simulink model "MMC_stack_openloop_NLM_CVB_dutycycleramp_twist"  (R2024b)
settings: Solver=FixedStepDiscrete  StartTime=t_init_sim  StopTime=sim_time  FixedStep=Ts  RelTol=1e-3
values from neighbouring files (symbols this model uses):
  a = 1    [param_stacksim_20260219.m]
  C1low1_active = 1    [script_MMC_stack_dutycycleramp_twist_20260219.m]
  C2low1_active = 1    [script_MMC_stack_dutycycleramp_twist_20260219.m]
  C_M_extra = C_m-twist_high_side_C    [param_stacksim_20260219.m]
  duty_cycle_max = 0.95    [script_MMC_stack_dutycycleramp_twist_20260219.m]
  duty_cycle_min = 0    [script_MMC_stack_dutycycleramp_twist_20260219.m]
  f0 = 50    [param_stacksim_20260219.m]
  feeder_current_lower_rate_limit = -10    [script_MMC_stack_dutycycleramp_twist_20260219.m]    (also in twist_parameters.m = -500)
  feeder_current_tab = [0.328 0.217 0.162 0.132 0.109 0.094 0.083 0.075 0.068 0.062 0.058 0.054 ... (42 elements, 14x3)]    [feeder_current.mat]
  feeder_current_upper_rate_limit = 0.386/(20e-3)    (= 19.3)    [twist_parameters.m]
  is6VExternallySupplied = true    [script_MMC_stack_dutycycleramp_twist_20260219.m]
  isDutyCycleRamp = true    [script_MMC_stack_dutycycleramp_twist_20260219.m]
  isFeederJumperOpen = true    [script_MMC_stack_dutycycleramp_twist_20260219.m]
  L_arm = 30e-3    (= 0.03)    [param_stacksim_20260219.m]
  m = 1    [param_stacksim_20260219.m]
  N = 5    [param_stacksim_20260219.m]
  power_losses = false    [script_MMC_stack_dutycycleramp_twist_20260219.m]
  R = 30    [param_stacksim_20260219.m]
  ramp_step_time = 500    [script_MMC_stack_dutycycleramp_twist_20260219.m]
  ramp_ticks = 4    [script_MMC_stack_dutycycleramp_twist_20260219.m]
  source_V = 0    [script_MMC_stack_dutycycleramp_twist_20260219.m]
  time_charge = 0.2    [script_MMC_stack_dutycycleramp_twist_20260219.m]
  time_decharge = 0.8    [script_MMC_stack_dutycycleramp_twist_20260219.m]
  Ts = 5e-7    (= 5e-07)    [script_MMC_stack_dutycycleramp_twist_20260219.m]
  twist_dead_time = 200e-9    (= 2e-07)    [twist_parameters.m]
  twist_freq_switching = 200e3    (= 200000)    [twist_parameters.m]
  twist_high_side_adc_R = 1/(1/2e6 + 1/2e6 + 1/(330e3+5.6e3))    (= 251272.836178)    [twist_parameters.m]
  twist_high_side_C = 33e-6*4 + 4.7e-6*12    (= 0.0001884)    [twist_parameters.m]
  twist_high_side_feeder_R = 47e3+4.7e3    (= 51700)    [twist_parameters.m]
  twist_high_side_rC = 0.1    [twist_parameters.m]
  twist_low_side_adc_R = 150e3+470    (= 150470)    [twist_parameters.m]
  twist_low_side_C_ceramic = 3*4.7e-6    (= 1.41e-05)    [twist_parameters.m]
  twist_low_side_C_electrolytic = 47e-6    (= 4.7e-05)    [twist_parameters.m]
  twist_low_side_L = 33e-6    (= 3.3e-05)    [twist_parameters.m]
  twist_low_side_rC = 700e-3    (= 0.7)    [twist_parameters.m]
  twist_low_side_rL = 20e-3    (= 0.02)    [twist_parameters.m]
  twist_R_VCC = (tau_VCC/twist_high_side_C  - twist_high_side_rC)/(1-(tau_VCC/twist_high_side_C - twist_high_side_rC)/R_parallel)    (= 1110.74997822)    [twist_parameters.m]
  VDC = 48    [param_stacksim_20260219.m]
undefined symbols (not defined in the file or in its folder): C_SM, feeder_current, gcbh, sps_rtmsupport, twist_data_acquisition_delay, twist_data_sampling_period, twist_low_side_lC
libraries: spsSeriesRLCBranchLib x66, spsTriangleGeneratorLib x30, spsMosfetLib x30, spsVoltageMeasurementLib x30, spsCurrentMeasurementLib x21, spsControlledCurrentSourceLib x15, spsDiodeLib x11, spsIdealSwitchLib x10, spsControlledVoltageSourceLib x1, spsGroundLib x1, spsMeanLib x1, spspowerguiLib x1
(part 1 of 9)
settings Model: Creator=ana  LastModifiedBy=ana

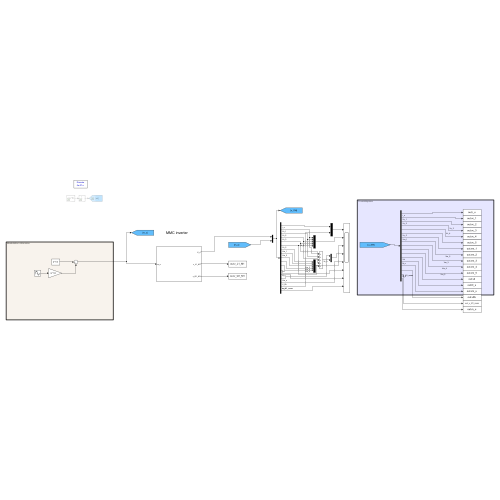
[thumbnail: Simulink's stored preview of the top-level diagram]
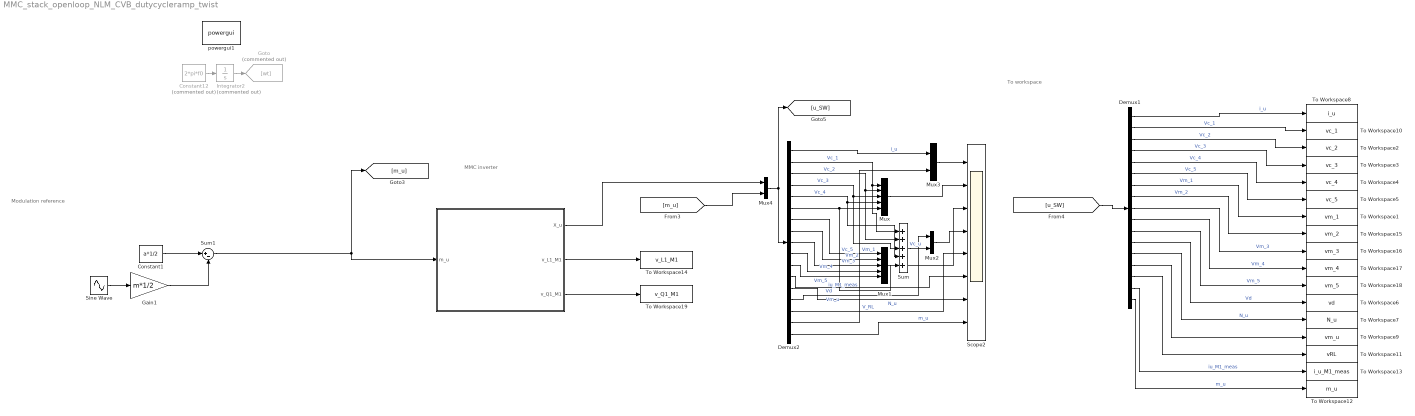
== system MMC_stack_openloop_NLM_CVB_dutycycleramp_twist ==
  note: MMC inverter
  note: To workspace
  note: Modulation reference
  " " : Subsystem
  Constant1 : Constant  Value=a*1/2
  Constant12 : Constant  Commented=on  Value=2*pi*f0
  Demux1 : Demux  Outputs=17
  Demux2 : Demux  Outputs=17
  Gain1 : Gain  Gain=m*1/2
  Goto : Goto  Commented=on  GotoTag=wt
  Integrator2 : Integrator  Commented=on
  Mux : Mux  Inputs=5
  Mux1 : Mux  Inputs=5
  Mux2 : Mux  Inputs=2
  Mux3 : Mux  Inputs=2
  Mux4 : Mux  Inputs=2
  Scope2 : Scope  NumInputPorts=8
  Sine Wave : Sin  Frequency=2*pi*f0  SampleTime=Ts
  Sum : Sum  Inputs=+++++
  Sum1 : Sum  Inputs=|+-
  To Workspace1 : ToWorkspace  VariableName=vm_1  SaveFormat=Structure With Time  SampleTime=-1
  To Workspace10 : ToWorkspace  VariableName=vc_1  SaveFormat=Structure With Time  SampleTime=-1
  To Workspace11 : ToWorkspace  VariableName=vRL  SaveFormat=Structure With Time  SampleTime=-1
  To Workspace12 : ToWorkspace  VariableName=m_u  SaveFormat=Structure With Time  SampleTime=-1
  To Workspace13 : ToWorkspace  VariableName=i_u_M1_meas  SaveFormat=Structure With Time  SampleTime=-1
  To Workspace14 : ToWorkspace  VariableName=v_L1_M1  SaveFormat=Structure With Time  SampleTime=-1
  To Workspace15 : ToWorkspace  VariableName=vm_2  SaveFormat=Structure With Time  SampleTime=-1
  To Workspace16 : ToWorkspace  VariableName=vm_3  SaveFormat=Structure With Time  SampleTime=-1
  To Workspace17 : ToWorkspace  VariableName=vm_4  SaveFormat=Structure With Time  SampleTime=-1
  To Workspace18 : ToWorkspace  VariableName=vm_5  SaveFormat=Structure With Time  SampleTime=-1
  To Workspace19 : ToWorkspace  VariableName=v_Q1_M1  SaveFormat=Structure With Time  SampleTime=-1
  To Workspace2 : ToWorkspace  VariableName=vc_2  SaveFormat=Structure With Time  SampleTime=-1
  To Workspace3 : ToWorkspace  VariableName=vc_3  SaveFormat=Structure With Time  SampleTime=-1
  To Workspace4 : ToWorkspace  VariableName=vc_4  SaveFormat=Structure With Time  SampleTime=-1
  To Workspace5 : ToWorkspace  VariableName=vc_5  SaveFormat=Structure With Time  SampleTime=-1
  To Workspace6 : ToWorkspace  VariableName=vd  SaveFormat=Structure With Time  SampleTime=-1
  To Workspace7 : ToWorkspace  VariableName=N_u  SaveFormat=Structure With Time  SampleTime=-1
  To Workspace8 : ToWorkspace  VariableName=i_u  SaveFormat=Structure With Time  SampleTime=-1
  To Workspace9 : ToWorkspace  VariableName=vm_u  SaveFormat=Structure With Time  SampleTime=-1
  powergui1 : spspowerguiLib/powergui  Priority=1  SimulationMode=Discrete  SampleTime=Ts  frequency=60  Iterations=50  frequencyindice=0  Pbase=100e6  ErrMax=1e-4  UnitsV=V  UnitsW=W  buscounter=0  FunctionMessages=off  echomessages=off  EnableUseOfTLC=off  CurrentSourceSwitches=off  DisableSnubberDevices=off  DisableRonSwitches=off  DisableVfSwitches=off  DisplayEquations=off  AutomaticDiscreteSolvers=off  SolverType=Backward Euler  Interpol=off  ExternalGateDelay=off  methode=off  Ts=0  x0status=blocks  SPID=off  SwTol=0  HookPort=off  NonlinearTolerance=1e-4  nMaxIteration=100  ContinueOnMaxIteration=off  RestoreLinks=warning  ResistiveCurrentMeasurement=off  Frange=[0:2:500]  Ylog=off  Xlog=on  ShowGrid=off  save=off  variable=ZData  structure=0  ZoomFFT=off  StartTime=0.0  cycles=1  DisplayStyle=1  fundamental=60  FreqAxis=off  MaxFrequency=1000  frequencyindicesteady=1  RmsSteady=1  display=off
  wires:
  Demux2/7 -> Mux1/1  "Vm_1"
  Demux2/11 -> Mux1/5  "Vm_5"
  Demux2/9 -> Mux1/3  "Vm_3"
  [u_SW] -> Demux1/1
  Demux1/8 -> To Workspace15/1  "Vm_2"
  Demux1/17 -> To Workspace12/1  "m_u"
  Demux2/10 -> Mux1/4  "Vm_4"
  Demux1/10 -> To Workspace17/1  "Vm_4"
  Demux1/5 -> To Workspace4/1  "Vc_4"
  Demux1/12 -> To Workspace6/1  "Vd"
  " "/1(X_u) -> Mux4/1
  Demux2/1 -> Mux3/1  "i_u"
  Constant1/1 -> Sum1/1
  Demux2/17 -> Scope2/8  "m_u"
  Demux1/11 -> To Workspace18/1  "Vm_5"
  [m_u] -> Mux4/2
  Demux2/6 -> Sum/5, Mux/5  "Vc_5"
  Mux4/1 -> [u_SW], Demux2/1
  Constant12/1 -> Integrator2/1
  Integrator2/1 -> Goto/1
  Demux1/9 -> To Workspace16/1  "Vm_3"
  Demux1/7 -> To Workspace1/1  "Vm_1"
  Demux1/3 -> To Workspace2/1  "Vc_2"
  Demux1/4 -> To Workspace3/1  "Vc_3"
  Demux1/6 -> To Workspace5/1  "Vc_5"
  Gain1/1 -> Sum1/2
  Demux1/2 -> To Workspace10/1  "Vc_1"
  Demux2/2 -> Sum/1, Mux/1  "Vc_1"
  Demux1/1 -> To Workspace8/1  "i_u"
  Demux2/5 -> Sum/4, Mux/4  "Vc_4"
  Demux2/3 -> Mux/2, Sum/2  "Vc_2"
  Demux2/4 -> Mux/3, Sum/3  "Vc_3"
  Mux/1 -> Scope2/2
  Demux2/8 -> Mux1/2  "Vm_2"
  Mux1/1 -> Scope2/3
  Demux2/13 -> Scope2/7  "N_u"
  Sum1/1 -> [m_u], " "/1(m_u)
  Demux2/12 -> Scope2/6  "Vd"
  Demux2/15 -> Scope2/5  "V_RL"
  Sum/1 -> Mux2/2  "Vc_u"
  Mux2/1 -> Scope2/4
  Demux2/14 -> Mux2/1  "Vm_u"
  Sine Wave/1 -> Gain1/1
  Demux1/13 -> To Workspace7/1  "N_u"
  Demux1/14 -> To Workspace9/1
  Demux1/15 -> To Workspace11/1
  Demux2/16 -> Mux3/2  "iu_M1_meas"
  Mux3/1 -> Scope2/1
  Demux1/16 -> To Workspace13/1  "iu_M1_meas"
  " "/2(v_L1_M1) -> To Workspace14/1
  " "/3(v_Q1_M1) -> To Workspace19/1

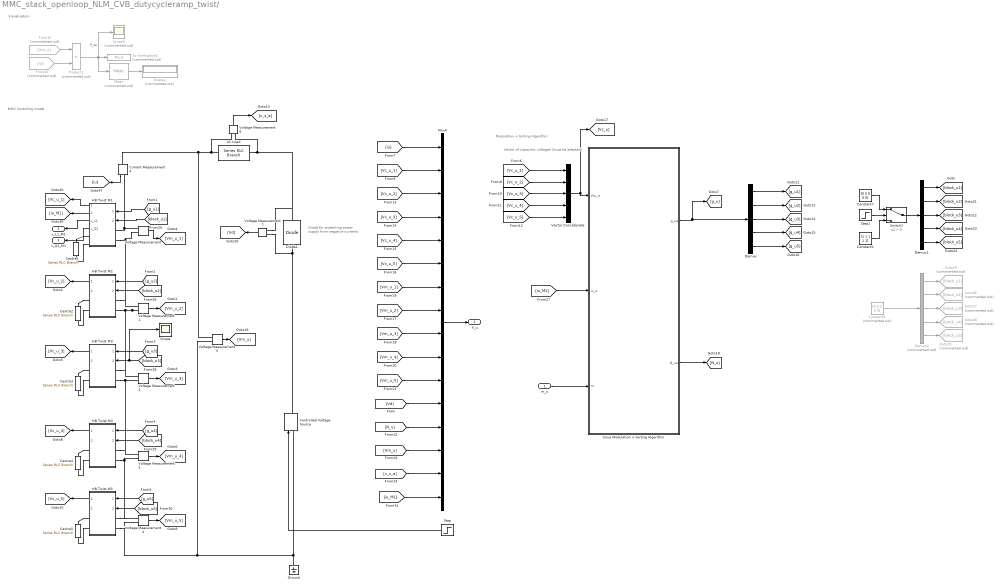
== system MMC_stack_openloop_NLM_CVB_dutycycleramp_twist/  ==
  note: Vector of capacitor voltages (must be adapted)
  note: Visualisation
  note: Modulation + Sorting Algorithm
  note: MMC Switching model
  note: Diode for protecting power supply from negative currents
  m_u : Inport
  AC Load : spsSeriesRLCBranchLib/Series RLC Branch  LConnTagsString=__new0  RConnTagsString=__new0  BranchType=R  Resistance=R  Inductance=L_arm  SetiL0=off  InitialCurrent=0  Capacitance=C_SM  Setx0=off  InitialVoltage=0  Measurements=None
  Cextra{1..5} (5 alike) : spsSeriesRLCBranchLib/Series RLC Branch  LConnTagsString=__new0  RConnTagsString=__new0  BranchType=C  Resistance=twist_high_side_rC  Inductance=1e-3  SetiL0=off  InitialCurrent=0  Capacitance=C_M_extra  Setx0=on  InitialVoltage=source_V  Measurements=None
  Constant2 : Constant  Value=[1 1 1 1 1]
  Constant3 : Constant  Commented=on  Value=[0 0 0 0 0]
  Constant7 : Constant  Value=[0 0 0 0 0]
  Controlled Voltage Source : spsControlledVoltageSourceLib/Controlled Voltage Source  Initialize=on  Source_Type=DC  Amplitude=VDC  Phase=0  Frequency=0  Measurements=None
  Current Measurement4 : spsCurrentMeasurementLib/Current Measurement  PhasorSimulation=off  OutputType=Complex  PSBequivalent=0
  Demux : Demux  Outputs=5
  Demux1 : Demux  Outputs=5
  Demux2 : Demux  Commented=on  Outputs=5
  Diode1 : spsDiodeLib/Diode  Ron=0.001  Lon=0  Vf=0.8  IC=0  UseSnubber=0  Rs=1e5  Cs=inf  Measurements=off
  Display : Display  Commented=on
  From32 : From  Commented=on  GotoTag=Vm_u
  From40 : From  Commented=on  GotoTag=iu
  Goto25 : Goto  Commented=on  GotoTag=block_u1
  Goto26 : Goto  Commented=on  GotoTag=block_u2
  Goto27 : Goto  Commented=on  GotoTag=block_u3
  Goto28 : Goto  Commented=on  GotoTag=block_u4
  Goto29 : Goto  Commented=on  GotoTag=block_u5
  Ground : spsGroundLib/Ground  LConnTagsString=a
  HB Twist M1 : Subsystem
  HB Twist M2 : Subsystem
  HB Twist M3 : Subsystem
  HB Twist M4 : Subsystem
  HB Twist M5 : Subsystem
  Mean : spsMeanLib/Mean  Commented=on  Freq=f0  Vinit=0  Ts=Ts
  Mux6 : Mux  Inputs=16
  Product1 : Product  Commented=on
  Scope : Scope
  Scope3 : Scope  Commented=on
  Sinus Modulation + Sorting Algorithm : Subsystem
  Step : Step  Time=time_decharge  Before=VDC  After=0  SampleTime=0
  Step1 : Step  Time=time_charge  SampleTime=Ts
  Switch1 : Switch  Criteria=u2 > Threshold  SaturateOnIntegerOverflow=off  InputSameDT=off
  To Workspace2 : ToWorkspace  Commented=on  VariableName=Pout  SaveFormat=Structure With Time  SampleTime=-1
  Vector Concatenate : Concatenate  NumInputs=5
  Voltage Measurement{,1..7} (8 alike) : spsVoltageMeasurementLib/Voltage Measurement  PhasorSimulation=off  OutputType=Complex  PSBequivalent=0
  X_u : Outport
  v_L1_M1 : Outport  Port=2
  v_Q1_M1 : Outport  Port=3
  wires:
  [Vc_u_1] -> Mux6/2
  Mux6/1 -> X_u/1
  Current Measurement4/1 -> [iu]
  Sinus Modulation + Sorting Algorithm/1(g_ua) -> Demux/1, [g_u]
  [iu_M1] -> Sinus Modulation + Sorting Algorithm/2(iu_a)
  Vector Concatenate/1 -> [Vc_u], Sinus Modulation + Sorting Algorithm/1(Vcu_a)
  m_u/1 -> Sinus Modulation + Sorting Algorithm/3(m)
  Product1/1 -> Mean/1, Scope3/1, To Workspace2/1  "P_sa"
  Voltage Measurement6/1 -> [v_s_a]
  From40/1 -> Product1/2
  HB Twist M1/1(v_High) -> [Vc_u_1]
  Voltage Measurement/1 -> [Vm_u_1]
  [g_u1] -> HB Twist M1/1(duty_cycle1)
  Voltage Measurement1/1 -> [Vm_u_2]
  HB Twist M2/1(v_High) -> [Vc_u_2]
  [g_u2] -> HB Twist M2/1(duty_cycle1)
  [g_u3] -> HB Twist M3/1(duty_cycle1)
  HB Twist M3/1(v_High) -> [Vc_u_3]
  Voltage Measurement2/1 -> [Vm_u_3]
  [g_u4] -> HB Twist M4/1(duty_cycle1)
  HB Twist M4/1(v_High) -> [Vc_u_4]
  Voltage Measurement3/1 -> [Vm_u_4]
  [g_u5] -> HB Twist M5/1(duty_cycle1)
  HB Twist M5/1(v_High) -> [Vc_u_5]
  Voltage Measurement4/1 -> [Vm_u_5]
  [Vc_u_1] -> Vector Concatenate/1
  [Vc_u_2] -> Vector Concatenate/2
  [Vc_u_3] -> Vector Concatenate/3
  [Vc_u_4] -> Vector Concatenate/4
  [Vc_u_5] -> Vector Concatenate/5
  Demux/1 -> [g_u1]
  Demux/2 -> [g_u2]
  Demux/3 -> [g_u3]
  Demux/4 -> [g_u4]
  Demux/5 -> [g_u5]
  [iu] -> Mux6/1
  [Vc_u_2] -> Mux6/3
  [Vc_u_3] -> Mux6/4
  [Vc_u_4] -> Mux6/5
  [Vc_u_5] -> Mux6/6
  [Vm_u_1] -> Mux6/7
  [Vm_u_2] -> Mux6/8
  [Vm_u_3] -> Mux6/9
  [Vm_u_4] -> Mux6/10
  [Vm_u_5] -> Mux6/11
  [Vd] -> Mux6/12
  Sinus Modulation + Sorting Algorithm/2(N_ua) -> [N_u]
  [N_u] -> Mux6/13
  Voltage Measurement5/1 -> [Vm_u]
  [Vm_u] -> Mux6/14
  [v_s_a] -> Mux6/15
  Voltage Measurement7/1 -> [Vd]
  Mean/1 -> Display/1
  [block_u1] -> HB Twist M1/2(block_leg1)
  [block_u2] -> HB Twist M2/2(block_leg1)
  [block_u3] -> HB Twist M3/2(block_leg1), Scope/1
  [block_u4] -> HB Twist M4/2(block_leg1)
  [block_u5] -> HB Twist M5/2(block_leg1)
  Step1/1 -> Switch1/2
  Switch1/1 -> Demux1/1
  Demux1/1 -> [block_u1]
  Demux1/2 -> [block_u2]
  Demux1/3 -> [block_u3]
  Demux1/4 -> [block_u4]
  Demux1/5 -> [block_u5]
  Constant7/1 -> Switch1/1
  Constant2/1 -> Switch1/3
  Demux2/3 -> Goto27/1
  Demux2/4 -> Goto28/1
  Constant3/1 -> Demux2/1
  Demux2/5 -> Goto29/1
  Demux2/2 -> Goto26/1
  Demux2/1 -> Goto25/1
  Step/1 -> Controlled Voltage Source/1
  HB Twist M1/2(i_1Low) -> [iu_M1]
  [iu_M1] -> Mux6/16
  From32/1 -> Product1/1
  HB Twist M1/3(v_L1) -> v_L1_M1/1
  HB Twist M1/4(v_Q1) -> v_Q1_M1/1
  connections:
  Voltage Measurement/LConn1 -- Current Measurement4/RConn1 -- HB Twist M1/LConn1
  Voltage Measurement6/LConn2 -- AC Load/RConn1 -- Voltage Measurement5/LConn1 -- Current Measurement4/LConn1
  Voltage Measurement3/LConn2 -- HB Twist M4/LConn2 -- HB Twist M5/LConn1 -- Voltage Measurement4/LConn1
  AC Load/LConn1 -- Diode1/RConn1 -- Voltage Measurement7/LConn1 -- Voltage Measurement6/LConn1
  HB Twist M1/LConn2 -- Voltage Measurement/LConn2 -- HB Twist M2/LConn1 -- Voltage Measurement1/LConn1
  Voltage Measurement2/LConn2 -- HB Twist M3/LConn2 -- HB Twist M4/LConn1 -- Voltage Measurement3/LConn1
  Voltage Measurement1/LConn2 -- HB Twist M2/LConn2 -- HB Twist M3/LConn1 -- Voltage Measurement2/LConn1
  HB Twist M5/LConn2 -- Voltage Measurement4/LConn2 -- Controlled Voltage Source/LConn1 -- Ground/LConn1 -- Voltage Measurement5/LConn2
  Voltage Measurement7/LConn2 -- Controlled Voltage Source/RConn1 -- Diode1/LConn1
  HB Twist M1/RConn1 -- Cextra1/LConn1
  HB Twist M1/RConn2 -- Cextra1/RConn1
  HB Twist M2/RConn1 -- Cextra2/LConn1
  HB Twist M2/RConn2 -- Cextra2/RConn1
  HB Twist M3/RConn1 -- Cextra3/LConn1
  HB Twist M3/RConn2 -- Cextra3/RConn1
  HB Twist M4/RConn1 -- Cextra4/LConn1
  HB Twist M4/RConn2 -- Cextra4/RConn1
  HB Twist M5/RConn1 -- Cextra5/LConn1
  HB Twist M5/RConn2 -- Cextra5/RConn1

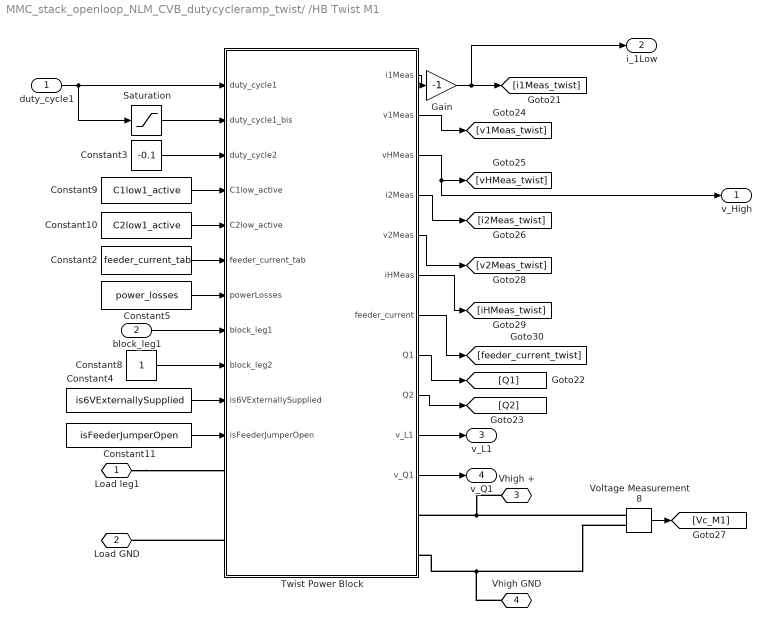
== system MMC_stack_openloop_NLM_CVB_dutycycleramp_twist/ /HB Twist M1 ==
  duty_cycle1 : Inport
  block_leg1 : Inport  Port=2
  Constant10 : Constant  Value=C2low1_active
  Constant11 : Constant  Value=isFeederJumperOpen
  Constant2 : Constant  Value=feeder_current_tab
  Constant3 : Constant  Value=-0.1
  Constant4 : Constant  Value=is6VExternallySupplied
  Constant5 : Constant  Value=power_losses
  Constant8 : Constant
  Constant9 : Constant  Value=C1low1_active
  Gain : Gain  Gain=-1
  Saturation : Saturate  UpperLimit=1  LowerLimit=0
  Twist Power Block : Subsystem
  Voltage Measurement8 : spsVoltageMeasurementLib/Voltage Measurement  PhasorSimulation=off  OutputType=Complex  PSBequivalent=0
  Load leg1 : PMIOPort  Side=Left
  Load GND : PMIOPort  Port=2  Side=Left
  Vhigh + : PMIOPort  Port=3  Side=Right
  Vhigh GND : PMIOPort  Port=4  Side=Right
  v_High : Outport
  i_1Low : Outport  Port=2
  v_L1 : Outport  Port=3
  v_Q1 : Outport  Port=4
  wires:
  duty_cycle1/1 -> Saturation/1, Twist Power Block/1(duty_cycle1)
  Twist Power Block/2(v1Meas) -> [v1Meas_twist]
  block_leg1/1 -> Twist Power Block/8(block_leg1)
  Constant4/1 -> Twist Power Block/10(is6VExternallySupplied)
  Constant5/1 -> Twist Power Block/7(powerLosses)
  Twist Power Block/1(i1Meas) -> Gain/1
  Twist Power Block/5(v2Meas) -> [v2Meas_twist]
  Constant10/1 -> Twist Power Block/5(C2low_active)
  Constant3/1 -> Twist Power Block/3(duty_cycle2)
  Constant11/1 -> Twist Power Block/11(isFeederJumperOpen)
  Twist Power Block/4(i2Meas) -> [i2Meas_twist]
  Twist Power Block/3(vHMeas) -> [vHMeas_twist], v_High/1
  Constant9/1 -> Twist Power Block/4(C1low_active)
  Twist Power Block/9(Q2) -> [Q2]
  Constant2/1 -> Twist Power Block/6(feeder_current_tab)
  Twist Power Block/6(iHMeas) -> [iHMeas_twist]
  Twist Power Block/7(feeder_current) -> [feeder_current_twist]
  Constant8/1 -> Twist Power Block/9(block_leg2)
  Twist Power Block/8(Q1) -> [Q1]
  Voltage Measurement8/1 -> [Vc_M1]
  Saturation/1 -> Twist Power Block/2(duty_cycle1_bis)
  Gain/1 -> i_1Low/1, [i1Meas_twist]
  Twist Power Block/10(v_L1) -> v_L1/1
  Twist Power Block/11(v_Q1) -> v_Q1/1
  connections:
  Voltage Measurement8/LConn2 -- Vhigh GND/RConn1 -- Twist Power Block/RConn2
  Voltage Measurement8/LConn1 -- Vhigh +/RConn1 -- Twist Power Block/RConn1
  Twist Power Block/LConn3 -- Load GND/RConn1
  Load leg1/RConn1 -- Twist Power Block/LConn1

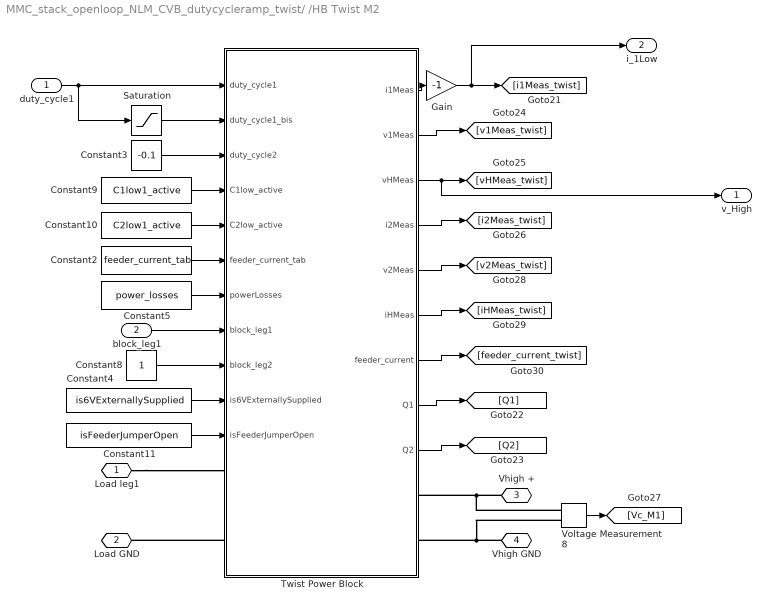
== system MMC_stack_openloop_NLM_CVB_dutycycleramp_twist/ /HB Twist M2 ==
  duty_cycle1 : Inport
  block_leg1 : Inport  Port=2
  Constant10 : Constant  Value=C2low1_active
  Constant11 : Constant  Value=isFeederJumperOpen
  Constant2 : Constant  Value=feeder_current_tab
  Constant3 : Constant  Value=-0.1
  Constant4 : Constant  Value=is6VExternallySupplied
  Constant5 : Constant  Value=power_losses
  Constant8 : Constant
  Constant9 : Constant  Value=C1low1_active
  Gain : Gain  Gain=-1
  Saturation : Saturate  UpperLimit=1  LowerLimit=0
  Twist Power Block : Subsystem
  Voltage Measurement8 : spsVoltageMeasurementLib/Voltage Measurement  PhasorSimulation=off  OutputType=Complex  PSBequivalent=0
  Load leg1 : PMIOPort  Side=Left
  Load GND : PMIOPort  Port=2  Side=Left
  Vhigh + : PMIOPort  Port=3  Side=Right
  Vhigh GND : PMIOPort  Port=4  Side=Right
  v_High : Outport
  i_1Low : Outport  Port=2
  wires:
  duty_cycle1/1 -> Saturation/1, Twist Power Block/1(duty_cycle1)
  Twist Power Block/2(v1Meas) -> [v1Meas_twist]
  block_leg1/1 -> Twist Power Block/8(block_leg1)
  Constant4/1 -> Twist Power Block/10(is6VExternallySupplied)
  Constant5/1 -> Twist Power Block/7(powerLosses)
  Twist Power Block/1(i1Meas) -> Gain/1
  Twist Power Block/5(v2Meas) -> [v2Meas_twist]
  Constant10/1 -> Twist Power Block/5(C2low_active)
  Constant3/1 -> Twist Power Block/3(duty_cycle2)
  Constant11/1 -> Twist Power Block/11(isFeederJumperOpen)
  Twist Power Block/4(i2Meas) -> [i2Meas_twist]
  Twist Power Block/3(vHMeas) -> [vHMeas_twist], v_High/1
  Constant9/1 -> Twist Power Block/4(C1low_active)
  Twist Power Block/9(Q2) -> [Q2]
  Constant2/1 -> Twist Power Block/6(feeder_current_tab)
  Twist Power Block/6(iHMeas) -> [iHMeas_twist]
  Twist Power Block/7(feeder_current) -> [feeder_current_twist]
  Constant8/1 -> Twist Power Block/9(block_leg2)
  Twist Power Block/8(Q1) -> [Q1]
  Voltage Measurement8/1 -> [Vc_M1]
  Saturation/1 -> Twist Power Block/2(duty_cycle1_bis)
  Gain/1 -> i_1Low/1, [i1Meas_twist]
  connections:
  Voltage Measurement8/LConn2 -- Vhigh GND/RConn1 -- Twist Power Block/RConn2
  Voltage Measurement8/LConn1 -- Vhigh +/RConn1 -- Twist Power Block/RConn1
  Twist Power Block/LConn3 -- Load GND/RConn1
  Load leg1/RConn1 -- Twist Power Block/LConn1

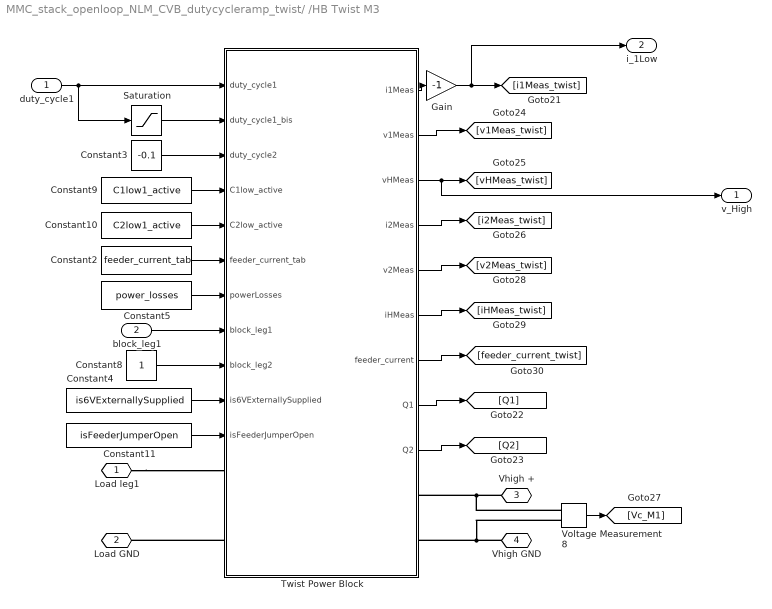
== system MMC_stack_openloop_NLM_CVB_dutycycleramp_twist/ /HB Twist M3 ==
  duty_cycle1 : Inport
  block_leg1 : Inport  Port=2
  Constant10 : Constant  Value=C2low1_active
  Constant11 : Constant  Value=isFeederJumperOpen
  Constant2 : Constant  Value=feeder_current_tab
  Constant3 : Constant  Value=-0.1
  Constant4 : Constant  Value=is6VExternallySupplied
  Constant5 : Constant  Value=power_losses
  Constant8 : Constant
  Constant9 : Constant  Value=C1low1_active
  Gain : Gain  Gain=-1
  Saturation : Saturate  UpperLimit=1  LowerLimit=0
  Twist Power Block : Subsystem
  Voltage Measurement8 : spsVoltageMeasurementLib/Voltage Measurement  PhasorSimulation=off  OutputType=Complex  PSBequivalent=0
  Load leg1 : PMIOPort  Side=Left
  Load GND : PMIOPort  Port=2  Side=Left
  Vhigh + : PMIOPort  Port=3  Side=Right
  Vhigh GND : PMIOPort  Port=4  Side=Right
  v_High : Outport
  i_1Low : Outport  Port=2
  wires:
  duty_cycle1/1 -> Saturation/1, Twist Power Block/1(duty_cycle1)
  Twist Power Block/2(v1Meas) -> [v1Meas_twist]
  block_leg1/1 -> Twist Power Block/8(block_leg1)
  Constant4/1 -> Twist Power Block/10(is6VExternallySupplied)
  Constant5/1 -> Twist Power Block/7(powerLosses)
  Twist Power Block/1(i1Meas) -> Gain/1
  Twist Power Block/5(v2Meas) -> [v2Meas_twist]
  Constant10/1 -> Twist Power Block/5(C2low_active)
  Constant3/1 -> Twist Power Block/3(duty_cycle2)
  Constant11/1 -> Twist Power Block/11(isFeederJumperOpen)
  Twist Power Block/4(i2Meas) -> [i2Meas_twist]
  Twist Power Block/3(vHMeas) -> [vHMeas_twist], v_High/1
  Constant9/1 -> Twist Power Block/4(C1low_active)
  Twist Power Block/9(Q2) -> [Q2]
  Constant2/1 -> Twist Power Block/6(feeder_current_tab)
  Twist Power Block/6(iHMeas) -> [iHMeas_twist]
  Twist Power Block/7(feeder_current) -> [feeder_current_twist]
  Constant8/1 -> Twist Power Block/9(block_leg2)
  Twist Power Block/8(Q1) -> [Q1]
  Voltage Measurement8/1 -> [Vc_M1]
  Saturation/1 -> Twist Power Block/2(duty_cycle1_bis)
  Gain/1 -> i_1Low/1, [i1Meas_twist]
  connections:
  Voltage Measurement8/LConn2 -- Vhigh GND/RConn1 -- Twist Power Block/RConn2
  Voltage Measurement8/LConn1 -- Vhigh +/RConn1 -- Twist Power Block/RConn1
  Twist Power Block/LConn3 -- Load GND/RConn1
  Load leg1/RConn1 -- Twist Power Block/LConn1

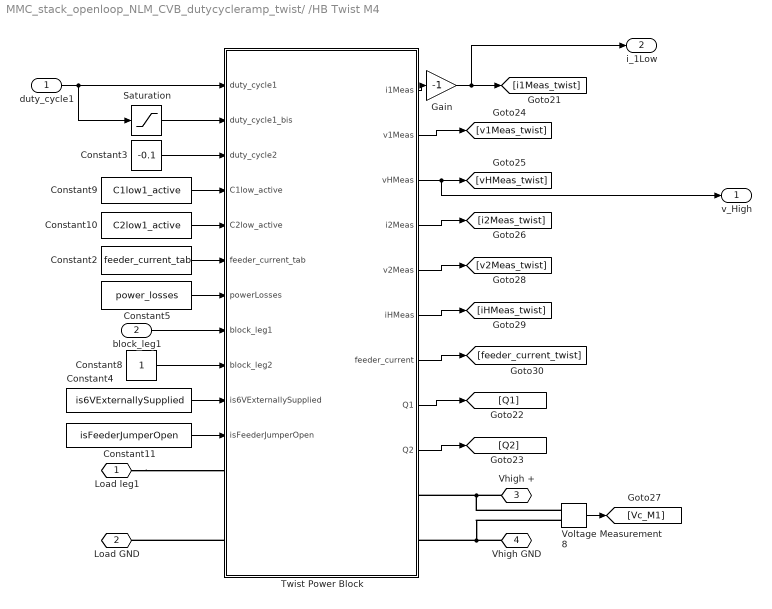
== system MMC_stack_openloop_NLM_CVB_dutycycleramp_twist/ /HB Twist M4 ==
  duty_cycle1 : Inport
  block_leg1 : Inport  Port=2
  Constant10 : Constant  Value=C2low1_active
  Constant11 : Constant  Value=isFeederJumperOpen
  Constant2 : Constant  Value=feeder_current_tab
  Constant3 : Constant  Value=-0.1
  Constant4 : Constant  Value=is6VExternallySupplied
  Constant5 : Constant  Value=power_losses
  Constant8 : Constant
  Constant9 : Constant  Value=C1low1_active
  Gain : Gain  Gain=-1
  Saturation : Saturate  UpperLimit=1  LowerLimit=0
  Twist Power Block : Subsystem
  Voltage Measurement8 : spsVoltageMeasurementLib/Voltage Measurement  PhasorSimulation=off  OutputType=Complex  PSBequivalent=0
  Load leg1 : PMIOPort  Side=Left
  Load GND : PMIOPort  Port=2  Side=Left
  Vhigh + : PMIOPort  Port=3  Side=Right
  Vhigh GND : PMIOPort  Port=4  Side=Right
  v_High : Outport
  i_1Low : Outport  Port=2
  wires:
  duty_cycle1/1 -> Saturation/1, Twist Power Block/1(duty_cycle1)
  Twist Power Block/2(v1Meas) -> [v1Meas_twist]
  block_leg1/1 -> Twist Power Block/8(block_leg1)
  Constant4/1 -> Twist Power Block/10(is6VExternallySupplied)
  Constant5/1 -> Twist Power Block/7(powerLosses)
  Twist Power Block/1(i1Meas) -> Gain/1
  Twist Power Block/5(v2Meas) -> [v2Meas_twist]
  Constant10/1 -> Twist Power Block/5(C2low_active)
  Constant3/1 -> Twist Power Block/3(duty_cycle2)
  Constant11/1 -> Twist Power Block/11(isFeederJumperOpen)
  Twist Power Block/4(i2Meas) -> [i2Meas_twist]
  Twist Power Block/3(vHMeas) -> [vHMeas_twist], v_High/1
  Constant9/1 -> Twist Power Block/4(C1low_active)
  Twist Power Block/9(Q2) -> [Q2]
  Constant2/1 -> Twist Power Block/6(feeder_current_tab)
  Twist Power Block/6(iHMeas) -> [iHMeas_twist]
  Twist Power Block/7(feeder_current) -> [feeder_current_twist]
  Constant8/1 -> Twist Power Block/9(block_leg2)
  Twist Power Block/8(Q1) -> [Q1]
  Voltage Measurement8/1 -> [Vc_M1]
  Saturation/1 -> Twist Power Block/2(duty_cycle1_bis)
  Gain/1 -> i_1Low/1, [i1Meas_twist]
  connections:
  Voltage Measurement8/LConn2 -- Vhigh GND/RConn1 -- Twist Power Block/RConn2
  Voltage Measurement8/LConn1 -- Vhigh +/RConn1 -- Twist Power Block/RConn1
  Twist Power Block/LConn3 -- Load GND/RConn1
  Load leg1/RConn1 -- Twist Power Block/LConn1

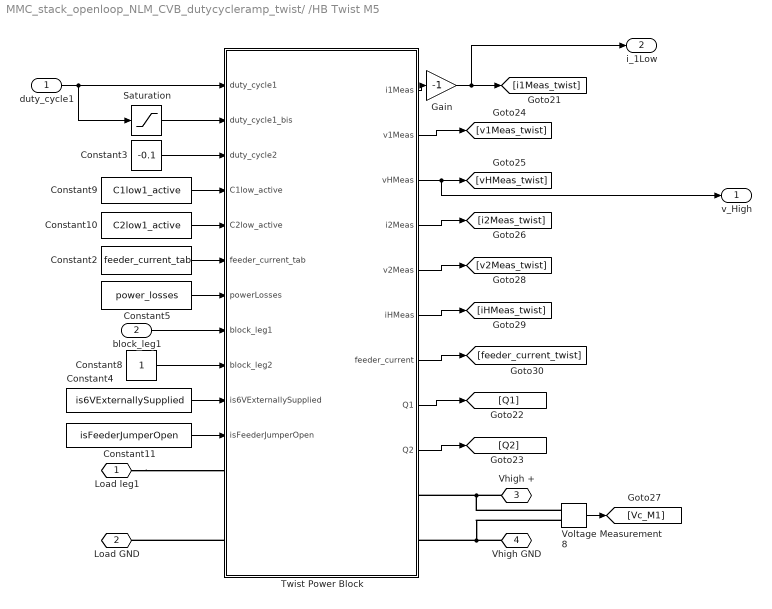
== system MMC_stack_openloop_NLM_CVB_dutycycleramp_twist/ /HB Twist M5 ==
  duty_cycle1 : Inport
  block_leg1 : Inport  Port=2
  Constant10 : Constant  Value=C2low1_active
  Constant11 : Constant  Value=isFeederJumperOpen
  Constant2 : Constant  Value=feeder_current_tab
  Constant3 : Constant  Value=-0.1
  Constant4 : Constant  Value=is6VExternallySupplied
  Constant5 : Constant  Value=power_losses
  Constant8 : Constant
  Constant9 : Constant  Value=C1low1_active
  Gain : Gain  Gain=-1
  Saturation : Saturate  UpperLimit=1  LowerLimit=0
  Twist Power Block : Subsystem
  Voltage Measurement8 : spsVoltageMeasurementLib/Voltage Measurement  PhasorSimulation=off  OutputType=Complex  PSBequivalent=0
  Load leg1 : PMIOPort  Side=Left
  Load GND : PMIOPort  Port=2  Side=Left
  Vhigh + : PMIOPort  Port=3  Side=Right
  Vhigh GND : PMIOPort  Port=4  Side=Right
  v_High : Outport
  i_1Low : Outport  Port=2
  wires:
  duty_cycle1/1 -> Saturation/1, Twist Power Block/1(duty_cycle1)
  Twist Power Block/2(v1Meas) -> [v1Meas_twist]
  block_leg1/1 -> Twist Power Block/8(block_leg1)
  Constant4/1 -> Twist Power Block/10(is6VExternallySupplied)
  Constant5/1 -> Twist Power Block/7(powerLosses)
  Twist Power Block/1(i1Meas) -> Gain/1
  Twist Power Block/5(v2Meas) -> [v2Meas_twist]
  Constant10/1 -> Twist Power Block/5(C2low_active)
  Constant3/1 -> Twist Power Block/3(duty_cycle2)
  Constant11/1 -> Twist Power Block/11(isFeederJumperOpen)
  Twist Power Block/4(i2Meas) -> [i2Meas_twist]
  Twist Power Block/3(vHMeas) -> [vHMeas_twist], v_High/1
  Constant9/1 -> Twist Power Block/4(C1low_active)
  Twist Power Block/9(Q2) -> [Q2]
  Constant2/1 -> Twist Power Block/6(feeder_current_tab)
  Twist Power Block/6(iHMeas) -> [iHMeas_twist]
  Twist Power Block/7(feeder_current) -> [feeder_current_twist]
  Constant8/1 -> Twist Power Block/9(block_leg2)
  Twist Power Block/8(Q1) -> [Q1]
  Voltage Measurement8/1 -> [Vc_M1]
  Saturation/1 -> Twist Power Block/2(duty_cycle1_bis)
  Gain/1 -> i_1Low/1, [i1Meas_twist]
  connections:
  Voltage Measurement8/LConn2 -- Vhigh GND/RConn1 -- Twist Power Block/RConn2
  Voltage Measurement8/LConn1 -- Vhigh +/RConn1 -- Twist Power Block/RConn1
  Twist Power Block/LConn3 -- Load GND/RConn1
  Load leg1/RConn1 -- Twist Power Block/LConn1

== system MMC_stack_openloop_NLM_CVB_dutycycleramp_twist/ /Sinus Modulation + Sorting Algorithm ==
  note: Phase A
  note: Verifies Non change
  Vcu_a : Inport
  iu_a : Inport  Port=2
  m : Inport  Port=3
  Constant : Constant
  Constant1 : Constant  Value=0
  Constant2 : Constant  Value=isDutyCycleRamp
  Constant3 : Constant  Value=-0.01
  GreaterThan : RelationalOperator  Operator=~=  OutDataTypeStr=boolean  RndMeth=Simplest  InputSameDT=off
  Memory : Memory  InheritSampleTime=on  LinearizeMemory=on  LinearizeAsDelay=on
  Number_of_Module_to_SWITCH : Subsystem
  Quantizer : Quantizer  QuantizationInterval=1/ramp_ticks
  Rate Limiter : RateLimiter  RisingSlewLimit=1/(ramp_step_time*1e-6)  FallingSlewLimit=-1/(ramp_step_time*1e-6)  SampleTimeMode=inherited  InitialCondition=-0.01
  Saturation : Saturate  UpperLimit=duty_cycle_max  LowerLimit=duty_cycle_min
  Saturation1 : Saturate  UpperLimit=duty_cycle_max  LowerLimit=duty_cycle_min
  Subsystem1 : Subsystem
      settings: PortSchema="{\"entries\":[{\"content\":{\"sides\":[{\"content\":{\"connectorIds\":[\"In1\",\"In2\",\"In3\"]},\"type\":\"ConnectorPlacement.EquallySpacedRectSide\",\"uuid\":\"25566ff9-210a-4488-8b15-702d65e93a4b\"},{\"content\":{\"connectorIds\":[\"Out1\"],\"side\":\"RIGHT\"},\"type\":\"ConnectorPlacement.EquallySpacedRectSide\",\"uuid\":\"97373fc2-3782-4e65-8804-644d53fa5380\"},{\"content\":{\"connectorIds\":[\"In4\"],\"side\":\"TOP\"},\"type\":\"ConnectorPlacement.EquallySpacedRectSide\",\"uuid\":\"e65d2433-d029-4e4a-b081-22e9ded4f272\"}]},\"type\":\"ConnectorPlacement.EquallySpacedConnector\",\"uuid\":\"235c80e7-78ad-4e69-a231-ec76d675b4ae\"}],\"packageUris\":[\"http://schema.mathworks.com/mf0/Connector/R2020b\"],\"version\":\"1.0\"}"
  Switch : Switch  Criteria=u2 > Threshold  SaturateOnIntegerOverflow=off  InputSameDT=off
  Switch1 : Switch  Criteria=u2 > Threshold  SaturateOnIntegerOverflow=off  InputSameDT=off
  Switch2 : Switch  Criteria=u2 > Threshold  SaturateOnIntegerOverflow=off  InputSameDT=off
  To Workspace1 : ToWorkspace  VariableName=g_u_after  SaveFormat=Structure With Time  SampleTime=-1
  To Workspace8 : ToWorkspace  VariableName=g_u_before  SaveFormat=Structure With Time  SampleTime=-1
  g_ua : Outport
  N_ua : Outport  Port=2
  wires:
  Vcu_a/1 -> Subsystem1/1(Vc_u)
  iu_a/1 -> Subsystem1/2(i_u)
  Number_of_Module_to_SWITCH/1(Nu_a) -> Subsystem1/3(N_on_u), GreaterThan/1, Memory/1, N_ua/1
  m/1 -> Number_of_Module_to_SWITCH/1(Modulante ua)
  Switch/1 -> Subsystem1/4(Pulse)
  Memory/1 -> GreaterThan/2
  GreaterThan/1 -> Switch/2
  Constant/1 -> Switch/1
  Constant1/1 -> Switch/3
  Constant2/1 -> Switch1/2
  Switch1/1 -> g_ua/1
  Saturation/1 -> Switch2/1
  Constant3/1 -> Switch2/3
  Quantizer/1 -> Saturation/1
  Rate Limiter/1 -> Switch2/2, Quantizer/1
  Saturation1/1 -> Switch1/3
  Switch2/1 -> To Workspace1/1, Switch1/1
  Subsystem1/1(g_u) -> To Workspace8/1, Rate Limiter/1, Saturation1/1

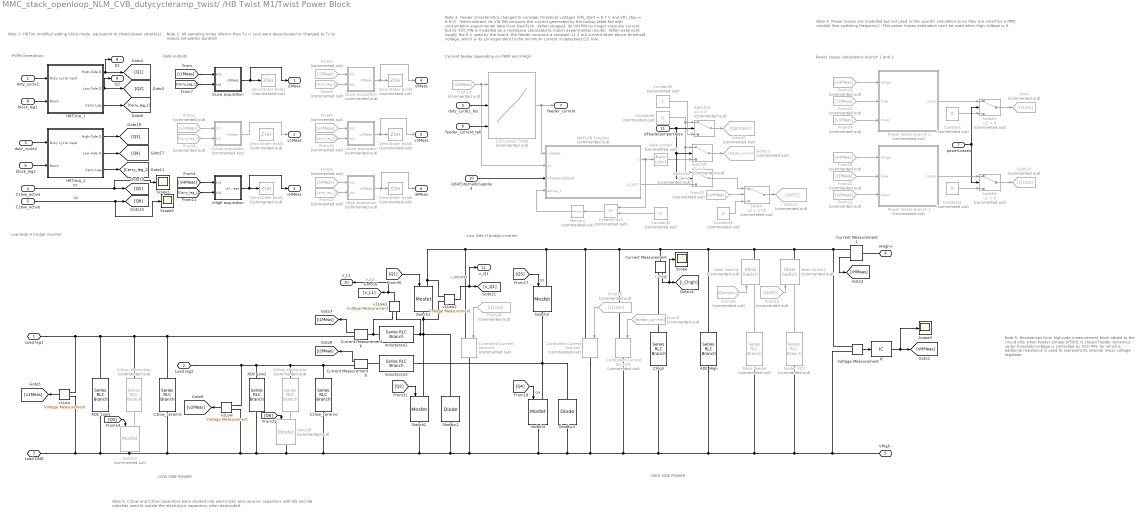
== system MMC_stack_openloop_NLM_CVB_dutycycleramp_twist/ /HB Twist M1/Twist Power Block ==
  note: Power losses calculations branch 1 and 2
  note: Current feeder depending on PWM and VHigh
  note: LOW SIDE POWER
  note: Data outputs
  note: PWM Generation
  note: Low-Side H bridge inverter
  note: Low Side H bridge inverter
  note: HIGH SIDE POWER
  note: Note 1:
      | HRTim modified adding block mode, equivalent to shield.power.stop(ALL);
  note: Note 2:
      | All sampling times inferior than Ts = 1e-6 were desactivated or changed to Ts to reduce simulation duration
  note: Note 3:
      | Feeder chracteristics changed to consider threshold voltages (Vth_start = 9.7 V and Vth_stop = 8.9 V).
      | -When started, its VIN PIN consums the current generated by the lookup table fed with consumption experimental data from OwnTech.
      | -When stopped, its VIN PIN no longer consums current but its VCC PIN is modelled as a resistance calculated to match experimental results.
      | -When externally supply the 6 V used by the board, the feeder consums a constant 11.2 mA current when above threshold voltage, which is its correspondent to the minimum current in datasheet (15 mA).
  note: Note 5:
      |
      | Resistances from high-side measurement block added to the circuit only when feeder jumper JP5001 is closed
      |
      | Feeder dynamics under threshold voltage is controlled by VCC PIN, for which a addtional resistance is used to represent its internal linear voltage regulator
  note: Note 4:
      | Power losses are modelled but not used in this specific simulation since they are small for a MMC module (low switching frequency).
      |
      | This power losses estimation can't be used when High voltage is 0.
  note: Note 6:
      | C1low and C2low capacitors were divided into electrolytic and ceramic capacitors with Q5 and Q6 switches used to isolate the electrolytic capacitors when demanded.
  duty_cycle1 : Inport
  duty_cycle1_bis : Inport  Port=2
  duty_cycle2 : Inport  Port=3
  C1low_active : Inport  Port=4
  C2low_active : Inport  Port=5
  feeder_current_tab : Inport  Port=6
  powerLosses : Inport  Port=7
  block_leg1 : Inport  Port=8
  block_leg2 : Inport  Port=9
  is6VExternallySupplied : Inport  Port=10
  isFeederJumperOpen : Inport  Port=11
  2-D Lookup Table : Lookup_n-D  Commented=on  LookupTableObject=feeder_current_tab  BreakpointsSpecification=Even spacing  BreakpointsForDimension1=[1:4]  BreakpointsForDimension2=[1:3]  BreakpointsForDimension1FirstPoint=feeder_VHigh_min  BreakpointsForDimension2FirstPoint=feeder_duty_min  BreakpointsForDimension1Spacing=feeder_VHigh_spacing  BreakpointsForDimension2Spacing=feeder_duty_spacing  TableSource=Input port  Table=feeder_current  InternalRulePriority=Speed  RndMeth=Simplest
      settings: InputPortMap=u0,u1,p221
  ADC High : spsSeriesRLCBranchLib/Series RLC Branch  LConnTagsString=__new0  RConnTagsString=__new0  BranchType=R  Resistance=twist_high_side_adc_R  Inductance=twist_low_side_L  SetiL0=off  InitialCurrent=0  Capacitance=1e-6  Setx0=off  InitialVoltage=0  Measurements=None
  ADC Low1 : spsSeriesRLCBranchLib/Series RLC Branch  LConnTagsString=__new0  RConnTagsString=__new0  BranchType=R  Resistance=twist_low_side_adc_R  Inductance=twist_low_side_L  SetiL0=off  InitialCurrent=0  Capacitance=1e-6  Setx0=off  InitialVoltage=0  Measurements=Branch voltage
  ADC Low2 : spsSeriesRLCBranchLib/Series RLC Branch  LConnTagsString=__new0  RConnTagsString=__new0  BranchType=R  Resistance=twist_low_side_adc_R  Inductance=twist_low_side_L  SetiL0=off  InitialCurrent=0  Capacitance=1e-6  Setx0=off  InitialVoltage=0  Measurements=Branch voltage
  C1low_ceramic : spsSeriesRLCBranchLib/Series RLC Branch  LConnTagsString=__new0  RConnTagsString=__new0  BranchType=C  Resistance=twist_low_side_rC  Inductance=1e-3  SetiL0=off  InitialCurrent=0  Capacitance=twist_low_side_C_ceramic  Setx0=off  InitialVoltage=source_V  Measurements=None
  C1low_electrolytic : spsSeriesRLCBranchLib/Series RLC Branch  Commented=on  LConnTagsString=__new0  RConnTagsString=__new0  BranchType=RC  Resistance=twist_low_side_rC  Inductance=twist_low_side_lC  SetiL0=off  InitialCurrent=0  Capacitance=twist_low_side_C_electrolytic  Setx0=off  InitialVoltage=source_V  Measurements=None
  C2low_ceramic : spsSeriesRLCBranchLib/Series RLC Branch  LConnTagsString=__new0  RConnTagsString=__new0  BranchType=C  Resistance=twist_low_side_rC  Inductance=1e-3  SetiL0=off  InitialCurrent=0  Capacitance=twist_low_side_C_ceramic  Setx0=off  InitialVoltage=source_V  Measurements=None
  C2low_electrolytic : spsSeriesRLCBranchLib/Series RLC Branch  Commented=on  LConnTagsString=__new0  RConnTagsString=__new0  BranchType=RC  Resistance=twist_low_side_rC  Inductance=twist_low_side_lC  SetiL0=off  InitialCurrent=0  Capacitance=twist_low_side_C_electrolytic  Setx0=off  InitialVoltage=source_V  Measurements=None
  Chigh : spsSeriesRLCBranchLib/Series RLC Branch  LConnTagsString=__new0  RConnTagsString=__new0  BranchType=RC  Resistance=twist_high_side_rC  Inductance=1e-3  SetiL0=off  InitialCurrent=0  Capacitance=twist_high_side_C  Setx0=on  InitialVoltage=source_V  Measurements=None
  Constant{,1..2,4,6} (5 alike) : Constant  Commented=on  Value=0
  Constant5 : Constant  Commented=on
  Controlled Current Source1 : spsControlledCurrentSourceLib/Controlled Current Source  Commented=on  Initialize=on  Source_Type=AC  Amplitude=0  Phase=0  Frequency=0  Measurements=None
  Controlled Current Source2 : spsControlledCurrentSourceLib/Controlled Current Source  Commented=on  Initialize=on  Source_Type=AC  Amplitude=0  Phase=0  Frequency=0  Measurements=None
  Controlled Current Source3 : spsControlledCurrentSourceLib/Controlled Current Source  Commented=on  Initialize=on  Source_Type=AC  Amplitude=0  Phase=0  Frequency=0  Measurements=None
  Current Measurement{,1,5..6} (4 alike) : spsCurrentMeasurementLib/Current Measurement  PhasorSimulation=off  OutputType=Complex  PSBequivalent=0
  From1 : From  Commented=on  GotoTag=v1Meas
  From10 : From  Commented=on  GotoTag=Carry_leg_2
  From12 : From  Commented=on  GotoTag=Carry_leg_2
  From{13,19..20,27} (4 alike) : From  Commented=on  GotoTag=vHMeas
  From15 : From  Commented=on  GotoTag=QVCC
  From16 : From  Commented=on  GotoTag=i2Loss
  From2 : From  Commented=on  GotoTag=i2Meas
  From21 : From  Commented=on  GotoTag=i2Meas
  From22 : From  Commented=on  GotoTag=v2Meas
  From23 : From  Commented=on  GotoTag=i1Meas
  From24 : From  Commented=on  GotoTag=v1Meas
  From26 : From  Commented=on  GotoTag=Qjumper
  From28 : From  Commented=on  GotoTag=i1Loss
  From4 : From  Commented=on  GotoTag=v2Meas
  From5 : From  Commented=on  GotoTag=iHMeas
  From6 : From  Commented=on  GotoTag=feeder_current
  From8 : From  Commented=on  GotoTag=Carry_leg_2
  From9 : From  Commented=on  GotoTag=Carry_leg_1
  Goto : Goto  Commented=on  GotoTag=i1Loss
  Goto12 : Goto  Commented=on  GotoTag=feeder_current
  Goto13 : Goto  Commented=on  GotoTag=QVCC
  Goto19 : Goto  Commented=on  GotoTag=i2Loss
  Goto20 : Goto  Commented=on  GotoTag=Qjumper
  GreaterThan : RelationalOperator  Commented=on  Operator=>  OutDataTypeStr=boolean  RndMeth=Simplest  InputSameDT=off
  HRTimA_1 : Subsystem
  HRTimA_2 : Subsystem
  IC : InitialCondition  Value=source_V
  Ideal Switch1 : spsIdealSwitchLib/Ideal Switch  Commented=on  Ron=0.001  Lon=0  IC=0  Rs=1e5  Cs=inf  Measurements=on
  Ideal Switch2 : spsIdealSwitchLib/Ideal Switch  Commented=on  Ron=0.001  Lon=0  IC=0  Rs=1e5  Cs=inf  Measurements=on
  Inductance1 : spsSeriesRLCBranchLib/Series RLC Branch  LConnTagsString=__new0  RConnTagsString=__new0  BranchType=RL  Resistance=twist_low_side_rL  Inductance=twist_low_side_L  SetiL0=off  InitialCurrent=0  Capacitance=1e-6  Setx0=off  InitialVoltage=0  Measurements=None
  Inductance2 : spsSeriesRLCBranchLib/Series RLC Branch  LConnTagsString=__new0  RConnTagsString=__new0  BranchType=RL  Resistance=twist_low_side_rL  Inductance=twist_low_side_L  SetiL0=off  InitialCurrent=0  Capacitance=1e-6  Setx0=off  InitialVoltage=0  Measurements=None
  MATLAB Function : MATLAB Function  Commented=on  TreatAsAtomicUnit=on
  Meas Feeder : spsSeriesRLCBranchLib/Series RLC Branch  Commented=on  LConnTagsString=__new0  RConnTagsString=__new0  BranchType=R  Resistance=twist_high_side_feeder_R  Inductance=twist_low_side_L  SetiL0=off  InitialCurrent=0  Capacitance=1e-6  Setx0=off  InitialVoltage=0  Measurements=None
  Memory : Memory  Commented=on  InheritSampleTime=on  LinearizeAsDelay=on
  Power losses branch 1 : Subsystem  Commented=on
  Power losses branch 2 : Subsystem  Commented=on
  Rate Limiter : RateLimiter  Commented=on  RisingSlewLimit=feeder_current_upper_rate_limit  FallingSlewLimit=feeder_current_lower_rate_limit  SampleTimeMode=inherited
  Scope{,1..3} (4 alike) : Scope
  Shottky2 : spsDiodeLib/Diode  Ron=twist_shottky_Ron  Lon=0  Vf=twist_shottky_Vf  IC=0  UseSnubber=0  Rs=twist_shottky_Rs  Cs=twist_shottky_Cs  Measurements=off
  Shottky4 : spsDiodeLib/Diode  Ron=twist_shottky_Ron  Lon=0  Vf=twist_shottky_Vf  IC=0  UseSnubber=0  Rs=twist_shottky_Rs  Cs=twist_shottky_Cs  Measurements=off
  Switch : Switch  Commented=on  Criteria=u2 > Threshold  Threshold=2.05  SaturateOnIntegerOverflow=off  InputSameDT=off
  Switch{1..4} (4 alike) : spsMosfetLib/Mosfet  Ron=twist_FET_Ron  Lon=0  Rd=twist_FET_Rd  Vfd=twist_FET_Vf  IC=0  Rs=twist_FET_Rs  Cs=twist_FET_Cs  Measurements=off
  Switch{5..6,9..11} (5 alike) : Switch  Commented=on  Criteria=u2 > Threshold  SaturateOnIntegerOverflow=off  InputSameDT=off
  Switch7 : spsMosfetLib/Mosfet  Commented=on  Ron=twist_FET_Clow_Ron  Lon=0  Rd=twist_FET_Clow_Rd  Vfd=twist_FET_Clow_Vf  IC=0  Rs=twist_FET_Rs  Cs=twist_FET_Cs  Measurements=off
  Switch8 : spsMosfetLib/Mosfet  Commented=on  Ron=twist_FET_Clow_Ron  Lon=0  Rd=twist_FET_Clow_Rd  Vfd=twist_FET_Clow_Vf  IC=0  Rs=twist_FET_Rs  Cs=twist_FET_Cs  Measurements=off
  Voltage Measurement : spsVoltageMeasurementLib/Voltage Measurement  PhasorSimulation=off  OutputType=Complex  PSBequivalent=0
  Zero-Order Hold{1..6} (6 alike) : ZeroOrderHold  Commented=on  SampleTime=twist_data_sampling_period
  feeder VCC : spsSeriesRLCBranchLib/Series RLC Branch  Commented=on  LConnTagsString=__new0  RConnTagsString=__new0  BranchType=R  Resistance=twist_R_VCC  Inductance=twist_low_side_L  SetiL0=off  InitialCurrent=0  Capacitance=1e-6  Setx0=off  InitialVoltage=0  Measurements=None
  i1Low acquisition : Subsystem
  i2Low acquisition : Subsystem  Commented=on
  iHigh acquisition : Subsystem  Commented=on
  v1Low : spsVoltageMeasurementLib/Voltage Measurement  PhasorSimulation=off  OutputType=Complex  PSBequivalent=0
  v1Low acquisition : Subsystem  Commented=on
  v1Low1 : spsVoltageMeasurementLib/Voltage Measurement  PhasorSimulation=off  OutputType=Complex  PSBequivalent=0
  v1Low2 : spsVoltageMeasurementLib/Voltage Measurement  PhasorSimulation=off  OutputType=Complex  PSBequivalent=0
  v2Low : spsVoltageMeasurementLib/Voltage Measurement  PhasorSimulation=off  OutputType=Complex  PSBequivalent=0
  v2Low acquisition : Subsystem  Commented=on
  vHigh acquisition : Subsystem
  Load leg1 : PMIOPort  Side=Left
  Load leg2 : PMIOPort  Port=2  Side=Left
  Load GND : PMIOPort  Port=3  Side=Left
  VHigh+ : PMIOPort  Port=4  Side=Right
  VHigh - : PMIOPort  Port=5  Side=Right
  i1Meas : Outport
  v1Meas : Outport  Port=2
  vHMeas : Outport  Port=3
  i2Meas : Outport  Port=4
  v2Meas : Outport  Port=5
  iHMeas : Outport  Port=6
  feeder_current : Outport  Port=7
  Q1 : Outport  Port=8
  Q2 : Outport  Port=9
  v_L1 : Outport  Port=10
  v_Q1 : Outport  Port=11
  wires:
  duty_cycle1/1 -> HRTimA_1/1(Duty cycle input)
  HRTimA_1/2(Low-Side Q) -> [Q2], Q2/1
  From1/1 -> v1Low acquisition/1(In1)
  C1low_active/1 -> Scope1/1, [Q5]  "Q5"
  HRTimA_1/1(High-Side Q) -> [Q1], Q1/1
  HRTimA_2/1(High-Side Q) -> [Q3]
  HRTimA_2/2(Low-Side Q) -> [Q4]
  [Carry_leg_1] -> vHigh acquisition/2(In2)
  [vHMeas] -> vHigh acquisition/1(In1)
  From2/1 -> i2Low acquisition/1(In1)
  From8/1 -> i2Low acquisition/2(In2)
  From4/1 -> v2Low acquisition/1(In1)
  From10/1 -> v2Low acquisition/2(In2)
  From5/1 -> iHigh acquisition/1(In1)
  From12/1 -> iHigh acquisition/2(In2)
  From9/1 -> v1Low acquisition/2(In2)
  v1Low acquisition/1(v1Meas) -> v1Meas/1
  i2Low acquisition/1(i2Meas) -> i2Meas/1, Zero-Order Hold4/1
  v2Low acquisition/1(v2Meas) -> v2Meas/1, Zero-Order Hold5/1
  iHigh acquisition/1(iHMeas) -> iHMeas/1, Zero-Order Hold6/1
  vHigh acquisition/1(vHMeas) -> Zero-Order Hold2/1, vHMeas/1
  HRTimA_2/3(Carry Leg) -> [Carry_leg_2]
  HRTimA_1/3(Carry Leg) -> [Carry_leg_1]
  duty_cycle2/1 -> HRTimA_2/1(Duty cycle input)
  From13/1 -> MATLAB Function/2(vC), 2-D Lookup Table/1
  v2Low/1 -> [v2Meas]
  [Q3] -> Switch3/1  "Q3"
  Current Measurement6/1 -> [i1Meas]
  [Q1] -> Switch1/1
  [Q4] -> Switch4/1  "Q4"
  v1Low/1 -> [v1Meas]
  [Q2] -> Switch2/1
  Current Measurement1/1 -> [iHMeas]
  Current Measurement5/1 -> [i2Meas]
  [Carry_leg_1] -> i1Low acquisition/2(In2)
  [i1Meas] -> i1Low acquisition/1(In1)
  Voltage Measurement/1 -> IC/1
  IC/1 -> Scope3/1, [vHMeas]
  From20/1 -> Power losses branch 1/1(VHigh)
  From23/1 -> Power losses branch 1/2(ILow)
  From24/1 -> Power losses branch 1/3(VLow)
  Power losses branch 1/1(i1Loss) -> Switch5/1
  Switch5/1 -> Goto/1
  Constant/1 -> Switch5/3
  feeder_current_tab/1 -> 2-D Lookup Table/3
  duty_cycle1_bis/1 -> 2-D Lookup Table/2
  [Q5] -> Switch7/1
  C2low_active/1 -> Scope2/1, [Q6]  "Q6"
  From6/1 -> Controlled Current Source1/1
  block_leg1/1 -> HRTimA_1/2(Block)
  Current Measurement/1 -> Scope/1, [i_Chigh]  "i_Chigh"
  block_leg2/1 -> HRTimA_2/2(Block)
  GreaterThan/1 -> Memory/1
  Constant2/1 -> GreaterThan/2
  From15/1 -> Ideal Switch2/1
  2-D Lookup Table/1 -> feeder_current/1, MATLAB Function/1(i_feeder)
  MATLAB Function/1(y) -> GreaterThan/1, Rate Limiter/1
  powerLosses/1 -> Switch5/2, Switch6/2
  From19/1 -> Power losses branch 2/1(VHigh)
  From21/1 -> Power losses branch 2/2(ILow)
  From22/1 -> Power losses branch 2/3(VLow)
  Switch6/1 -> Goto19/1
  Constant1/1 -> Switch6/3
  Power losses branch 2/1(i1Loss) -> Switch6/1
  is6VExternallySupplied/1 -> MATLAB Function/3(isfeederdisabled)
  Memory/1 -> MATLAB Function/4(active_1)
  From27/1 -> Switch/2
  Constant4/1 -> Switch/3
  [Q6] -> Switch8/1
  Switch9/1 -> Goto12/1
  Rate Limiter/1 -> Switch9/3
  MATLAB Function/2(Q_VCC) -> Switch10/3
  Constant6/1 -> Switch11/1, Switch10/1, Switch9/1
  isFeederJumperOpen/1 -> Switch11/2, Switch9/2, Switch10/2
  Switch/1 -> Goto13/1
  Switch10/1 -> Switch/1
  Constant5/1 -> Switch11/3
  Switch11/1 -> Goto20/1
  From26/1 -> Ideal Switch1/1
  From16/1 -> Controlled Current Source2/1
  From28/1 -> Controlled Current Source3/1
  i1Low acquisition/1(i1Meas) -> Zero-Order Hold1/1, i1Meas/1
  v1Low1/1 -> v_L1/1, [v_L1]  "v_L1"
  v1Low2/1 -> v_Q1/1, [v_Q1]  "v_MOSFET"
  connections:
  Inductance2/LConn1 -- Current Measurement5/LConn1
  Current Measurement6/LConn1 -- v1Low1/LConn2 -- Inductance1/LConn1
  VHigh+/RConn1 -- Current Measurement1/LConn1
  v2Low/LConn1 -- Load leg2/RConn1 -- ADC Low2/LConn1 -- C2low_electrolytic/LConn1 -- C2low_ceramic/LConn1 -- Current Measurement5/RConn1
  Switch4/LConn1 -- Switch3/RConn1 -- Shottky4/RConn1 -- Inductance2/RConn1
  v1Low/LConn1 -- Load leg1/RConn1 -- C1low_ceramic/LConn1 -- Current Measurement6/RConn1 -- C1low_electrolytic/LConn1 -- ADC Low1/LConn1
  Current Measurement/RConn1 -- Chigh/LConn1
  ADC High/RConn1 -- Meas Feeder/RConn1 -- feeder VCC/RConn1 -- Voltage Measurement/LConn2 -- VHigh -/RConn1 -- Chigh/RConn1 -- Controlled Current Source2/RConn1 -- Controlled Current Source3/RConn1 -- Switch2/RConn1 -- Load GND/RConn1 -- v1Low/LConn2 -- ADC Low1/RConn1 -- Switch7/RConn1 -- C1low_ceramic/RConn1 -- v2Low/LConn2 -- ADC Low2/RConn1 -- Switch8/RConn1 -- C2low_ceramic/RConn1 -- Shottky2/LConn1 -- Switch4/RConn1 -- Shottky4/LConn1 -- Controlled Current Source1/RConn1
  Switch7/LConn1 -- C1low_electrolytic/RConn1
  Switch8/LConn1 -- C2low_electrolytic/RConn1
  Inductance1/RConn1 -- v1Low1/LConn1 -- v1Low2/LConn2 -- Switch1/RConn1 -- Shottky2/RConn1 -- Switch2/LConn1
  Ideal Switch2/LConn1 -- feeder VCC/LConn1
  Current Measurement/LConn1 -- Ideal Switch1/RConn1 -- Voltage Measurement/LConn1 -- Current Measurement1/RConn1 -- Ideal Switch2/RConn1 -- ADC High/LConn1 -- Controlled Current Source2/LConn1 -- Controlled Current Source3/LConn1 -- v1Low2/LConn1 -- Switch1/LConn1 -- Switch3/LConn1 -- Controlled Current Source1/LConn1
  Meas Feeder/LConn1 -- Ideal Switch1/LConn1
